simulink model "sm_car"  (R2025a)
settings: Solver=ode23t  StartTime=0.0  StopTime=400  MaxStep=0.4  RelTol=1e-3  AbsTol=1e-3  EnableMultiTasking=on
PreLoadFcn:
  | % Due to usability issue in Repeating Sequence block
  | warning('off','Simulink:Masking:Invalid');
  | 
  | % Eliminate unnecessary warnings in inactive variants
  | % Warnings generated only if you click through inactive variant
  | warning('off','MATLAB:nonExistentField');
  | warning('off','Simulink:Parameters:BlkParamUndefined');
PostLoadFcn:
  | set_param([bdroot '/Vehicle'],'popup_trailer','Off')
  | warning('off','sm:sli:setup:compile:LocalSolverNotSupported')
  | %sm_car_config_maneuver(bdroot,'WOT Braking');
  | sm_car_config_vehicle(bdroot,'false');
  | sm_car_config_logging(bdroot);
InitFcn:
  | sm_car_config_camera;
  | Vehicle = sm_car_vehcfg_checkConfig(Vehicle);
  | sm_car_check_tire_model(bdroot);
StartFcn:
  | tic;
StopFcn:
  | Elapsed_Sim_Time = toc;
  | % disp(['Elapsed Sim Time = ' num2str(Elapsed_Sim_Time)]);
undefined symbols (not defined in the file): Axle1D, AxleIn, Camera, Control, Driver, Free, Init, Maneuver, Pedal, RaceFix, RaceSpin, Scene, ShaftL1, ShaftL2, ShaftR1, ShaftR2, Soft, Stiff, Visual, X, xy_data_car_side, Y, Z
libraries: sm_lib x1546, nesl_utility x528, fl_lib x480, SimscapeFluids_lib x61, sdl_lib x49, simulink x29, ee_lib x7, simulink_extras x6, Linkage_Systems x4, Tire_1x2x x4, AntiRollBar_Systems x2, Linkage_Decoupled x2
(part 3 of 79)

== system sm_car/Camera Frames/Transform FR ==
  Transform Camera Frame : sm_lib/Frames and Transforms/Rigid Transform  RotationMethod=RotationSequence  FollAlignAxisA=+X  BaseAlignAxisA=+Y  FollAlignAxisB=+Y  BaseAlignAxisB=+Z  RotationStandardAxis=+Z  RotationAngle=0.0  RotationAngleUnits=deg  RotationArbitraryAxis=[0 0 1]  RotationSequenceAxes=FollowerAxes  RotationSequence=ZYX  RotationSequenceAngles=CF.a.Value(3:-1:1)  RotationSequenceAnglesUnits=deg  RotationMatrix=[1 0 0; 0 1 0; 0 0 1]  Quaternion=[1 0 0 0]  TranslationMethod=Cartesian  TranslationCartesianOffset=CF.s.Value  TranslationCartesianOffsetUnits=m  TranslationStandardAxis=+Z  TranslationStandardOffset=0  TranslationStandardOffsetUnits=m  TranslationROffset=0  TranslationROffsetUnits=m  TranslationThetaOffset=0  TranslationThetaOffsetUnits=deg  TranslationZOffset=0  TranslationZOffsetUnits=m
  B : PMIOPort  Side=Left
  F : PMIOPort  Port=2  Side=Right
  connections:
  Transform Camera Frame/RConn1 -- F/RConn1
  Transform Camera Frame/LConn1 -- B/RConn1

== system sm_car/Camera Frames/Transform FixO FL ==
  Transform Camera Frame : sm_lib/Frames and Transforms/Rigid Transform  RotationMethod=RotationSequence  FollAlignAxisA=+X  BaseAlignAxisA=+Y  FollAlignAxisB=+Y  BaseAlignAxisB=+Z  RotationStandardAxis=+Z  RotationAngle=0.0  RotationAngleUnits=deg  RotationArbitraryAxis=[0 0 1]  RotationSequenceAxes=FollowerAxes  RotationSequence=ZYX  RotationSequenceAngles=CF.a.Value(3:-1:1)  RotationSequenceAnglesUnits=deg  RotationMatrix=[1 0 0; 0 1 0; 0 0 1]  Quaternion=[1 0 0 0]  TranslationMethod=Cartesian  TranslationCartesianOffset=CF.s.Value  TranslationCartesianOffsetUnits=m  TranslationStandardAxis=+Z  TranslationStandardOffset=0  TranslationStandardOffsetUnits=m  TranslationROffset=0  TranslationROffsetUnits=m  TranslationThetaOffset=0  TranslationThetaOffsetUnits=deg  TranslationZOffset=0  TranslationZOffsetUnits=m
  B : PMIOPort  Side=Left
  F : PMIOPort  Port=2  Side=Right
  connections:
  Transform Camera Frame/RConn1 -- F/RConn1
  Transform Camera Frame/LConn1 -- B/RConn1

== system sm_car/Camera Frames/Transform FixO FR ==
  Transform Camera Frame : sm_lib/Frames and Transforms/Rigid Transform  RotationMethod=RotationSequence  FollAlignAxisA=+X  BaseAlignAxisA=+Y  FollAlignAxisB=+Y  BaseAlignAxisB=+Z  RotationStandardAxis=+Z  RotationAngle=0.0  RotationAngleUnits=deg  RotationArbitraryAxis=[0 0 1]  RotationSequenceAxes=FollowerAxes  RotationSequence=ZYX  RotationSequenceAngles=CF.a.Value(3:-1:1)  RotationSequenceAnglesUnits=deg  RotationMatrix=[1 0 0; 0 1 0; 0 0 1]  Quaternion=[1 0 0 0]  TranslationMethod=Cartesian  TranslationCartesianOffset=CF.s.Value  TranslationCartesianOffsetUnits=m  TranslationStandardAxis=+Z  TranslationStandardOffset=0  TranslationStandardOffsetUnits=m  TranslationROffset=0  TranslationROffsetUnits=m  TranslationThetaOffset=0  TranslationThetaOffsetUnits=deg  TranslationZOffset=0  TranslationZOffsetUnits=m
  B : PMIOPort  Side=Left
  F : PMIOPort  Port=2  Side=Right
  connections:
  Transform Camera Frame/RConn1 -- F/RConn1
  Transform Camera Frame/LConn1 -- B/RConn1

== system sm_car/Camera Frames/Transform FixO Front ==
  Transform Camera Frame : sm_lib/Frames and Transforms/Rigid Transform  RotationMethod=RotationSequence  FollAlignAxisA=+X  BaseAlignAxisA=+Y  FollAlignAxisB=+Y  BaseAlignAxisB=+Z  RotationStandardAxis=+Z  RotationAngle=0.0  RotationAngleUnits=deg  RotationArbitraryAxis=[0 0 1]  RotationSequenceAxes=FollowerAxes  RotationSequence=ZYX  RotationSequenceAngles=CF.a.Value(3:-1:1)  RotationSequenceAnglesUnits=deg  RotationMatrix=[1 0 0; 0 1 0; 0 0 1]  Quaternion=[1 0 0 0]  TranslationMethod=Cartesian  TranslationCartesianOffset=CF.s.Value  TranslationCartesianOffsetUnits=m  TranslationStandardAxis=+Z  TranslationStandardOffset=0  TranslationStandardOffsetUnits=m  TranslationROffset=0  TranslationROffsetUnits=m  TranslationThetaOffset=0  TranslationThetaOffsetUnits=deg  TranslationZOffset=0  TranslationZOffsetUnits=m
  B : PMIOPort  Side=Left
  F : PMIOPort  Port=2  Side=Right
  connections:
  Transform Camera Frame/RConn1 -- F/RConn1
  Transform Camera Frame/LConn1 -- B/RConn1

== system sm_car/Camera Frames/Transform FixO Left ==
  Transform Camera Frame : sm_lib/Frames and Transforms/Rigid Transform  RotationMethod=RotationSequence  FollAlignAxisA=+X  BaseAlignAxisA=+Y  FollAlignAxisB=+Y  BaseAlignAxisB=+Z  RotationStandardAxis=+Z  RotationAngle=0.0  RotationAngleUnits=deg  RotationArbitraryAxis=[0 0 1]  RotationSequenceAxes=FollowerAxes  RotationSequence=ZYX  RotationSequenceAngles=CF.a.Value(3:-1:1)  RotationSequenceAnglesUnits=deg  RotationMatrix=[1 0 0; 0 1 0; 0 0 1]  Quaternion=[1 0 0 0]  TranslationMethod=Cartesian  TranslationCartesianOffset=CF.s.Value  TranslationCartesianOffsetUnits=m  TranslationStandardAxis=+Z  TranslationStandardOffset=0  TranslationStandardOffsetUnits=m  TranslationROffset=0  TranslationROffsetUnits=m  TranslationThetaOffset=0  TranslationThetaOffsetUnits=deg  TranslationZOffset=0  TranslationZOffsetUnits=m
  B : PMIOPort  Side=Left
  F : PMIOPort  Port=2  Side=Right
  connections:
  Transform Camera Frame/RConn1 -- F/RConn1
  Transform Camera Frame/LConn1 -- B/RConn1

== system sm_car/Camera Frames/Transform FixO RL ==
  Transform Camera Frame : sm_lib/Frames and Transforms/Rigid Transform  RotationMethod=RotationSequence  FollAlignAxisA=+X  BaseAlignAxisA=+Y  FollAlignAxisB=+Y  BaseAlignAxisB=+Z  RotationStandardAxis=+Z  RotationAngle=0.0  RotationAngleUnits=deg  RotationArbitraryAxis=[0 0 1]  RotationSequenceAxes=FollowerAxes  RotationSequence=ZYX  RotationSequenceAngles=CF.a.Value(3:-1:1)  RotationSequenceAnglesUnits=deg  RotationMatrix=[1 0 0; 0 1 0; 0 0 1]  Quaternion=[1 0 0 0]  TranslationMethod=Cartesian  TranslationCartesianOffset=CF.s.Value  TranslationCartesianOffsetUnits=m  TranslationStandardAxis=+Z  TranslationStandardOffset=0  TranslationStandardOffsetUnits=m  TranslationROffset=0  TranslationROffsetUnits=m  TranslationThetaOffset=0  TranslationThetaOffsetUnits=deg  TranslationZOffset=0  TranslationZOffsetUnits=m
  B : PMIOPort  Side=Left
  F : PMIOPort  Port=2  Side=Right
  connections:
  Transform Camera Frame/RConn1 -- F/RConn1
  Transform Camera Frame/LConn1 -- B/RConn1

== system sm_car/Camera Frames/Transform FixO RR ==
  Transform Camera Frame : sm_lib/Frames and Transforms/Rigid Transform  RotationMethod=RotationSequence  FollAlignAxisA=+X  BaseAlignAxisA=+Y  FollAlignAxisB=+Y  BaseAlignAxisB=+Z  RotationStandardAxis=+Z  RotationAngle=0.0  RotationAngleUnits=deg  RotationArbitraryAxis=[0 0 1]  RotationSequenceAxes=FollowerAxes  RotationSequence=ZYX  RotationSequenceAngles=CF.a.Value(3:-1:1)  RotationSequenceAnglesUnits=deg  RotationMatrix=[1 0 0; 0 1 0; 0 0 1]  Quaternion=[1 0 0 0]  TranslationMethod=Cartesian  TranslationCartesianOffset=CF.s.Value  TranslationCartesianOffsetUnits=m  TranslationStandardAxis=+Z  TranslationStandardOffset=0  TranslationStandardOffsetUnits=m  TranslationROffset=0  TranslationROffsetUnits=m  TranslationThetaOffset=0  TranslationThetaOffsetUnits=deg  TranslationZOffset=0  TranslationZOffsetUnits=m
  B : PMIOPort  Side=Left
  F : PMIOPort  Port=2  Side=Right
  connections:
  Transform Camera Frame/RConn1 -- F/RConn1
  Transform Camera Frame/LConn1 -- B/RConn1

== system sm_car/Camera Frames/Transform FixO Rear ==
  Transform Camera Frame : sm_lib/Frames and Transforms/Rigid Transform  RotationMethod=RotationSequence  FollAlignAxisA=+X  BaseAlignAxisA=+Y  FollAlignAxisB=+Y  BaseAlignAxisB=+Z  RotationStandardAxis=+Z  RotationAngle=0.0  RotationAngleUnits=deg  RotationArbitraryAxis=[0 0 1]  RotationSequenceAxes=FollowerAxes  RotationSequence=ZYX  RotationSequenceAngles=CF.a.Value(3:-1:1)  RotationSequenceAnglesUnits=deg  RotationMatrix=[1 0 0; 0 1 0; 0 0 1]  Quaternion=[1 0 0 0]  TranslationMethod=Cartesian  TranslationCartesianOffset=CF.s.Value  TranslationCartesianOffsetUnits=m  TranslationStandardAxis=+Z  TranslationStandardOffset=0  TranslationStandardOffsetUnits=m  TranslationROffset=0  TranslationROffsetUnits=m  TranslationThetaOffset=0  TranslationThetaOffsetUnits=deg  TranslationZOffset=0  TranslationZOffsetUnits=m
  B : PMIOPort  Side=Left
  F : PMIOPort  Port=2  Side=Right
  connections:
  Transform Camera Frame/RConn1 -- F/RConn1
  Transform Camera Frame/LConn1 -- B/RConn1

== system sm_car/Camera Frames/Transform FixO Right ==
  Transform Camera Frame : sm_lib/Frames and Transforms/Rigid Transform  RotationMethod=RotationSequence  FollAlignAxisA=+X  BaseAlignAxisA=+Y  FollAlignAxisB=+Y  BaseAlignAxisB=+Z  RotationStandardAxis=+Z  RotationAngle=0.0  RotationAngleUnits=deg  RotationArbitraryAxis=[0 0 1]  RotationSequenceAxes=FollowerAxes  RotationSequence=ZYX  RotationSequenceAngles=CF.a.Value(3:-1:1)  RotationSequenceAnglesUnits=deg  RotationMatrix=[1 0 0; 0 1 0; 0 0 1]  Quaternion=[1 0 0 0]  TranslationMethod=Cartesian  TranslationCartesianOffset=CF.s.Value  TranslationCartesianOffsetUnits=m  TranslationStandardAxis=+Z  TranslationStandardOffset=0  TranslationStandardOffsetUnits=m  TranslationROffset=0  TranslationROffsetUnits=m  TranslationThetaOffset=0  TranslationThetaOffsetUnits=deg  TranslationZOffset=0  TranslationZOffsetUnits=m
  B : PMIOPort  Side=Left
  F : PMIOPort  Port=2  Side=Right
  connections:
  Transform Camera Frame/RConn1 -- F/RConn1
  Transform Camera Frame/LConn1 -- B/RConn1

== system sm_car/Camera Frames/Transform FixO Top ==
  Transform Camera Frame : sm_lib/Frames and Transforms/Rigid Transform  RotationMethod=RotationSequence  FollAlignAxisA=+X  BaseAlignAxisA=+Y  FollAlignAxisB=+Y  BaseAlignAxisB=+Z  RotationStandardAxis=+Z  RotationAngle=0.0  RotationAngleUnits=deg  RotationArbitraryAxis=[0 0 1]  RotationSequenceAxes=FollowerAxes  RotationSequence=ZYX  RotationSequenceAngles=CF.a.Value(3:-1:1)  RotationSequenceAnglesUnits=deg  RotationMatrix=[1 0 0; 0 1 0; 0 0 1]  Quaternion=[1 0 0 0]  TranslationMethod=Cartesian  TranslationCartesianOffset=CF.s.Value  TranslationCartesianOffsetUnits=m  TranslationStandardAxis=+Z  TranslationStandardOffset=0  TranslationStandardOffsetUnits=m  TranslationROffset=0  TranslationROffsetUnits=m  TranslationThetaOffset=0  TranslationThetaOffsetUnits=deg  TranslationZOffset=0  TranslationZOffsetUnits=m
  B : PMIOPort  Side=Left
  F : PMIOPort  Port=2  Side=Right
  connections:
  Transform Camera Frame/RConn1 -- F/RConn1
  Transform Camera Frame/LConn1 -- B/RConn1

== system sm_car/Camera Frames/Transform Front ==
  Transform Camera Frame : sm_lib/Frames and Transforms/Rigid Transform  RotationMethod=RotationSequence  FollAlignAxisA=+X  BaseAlignAxisA=+Y  FollAlignAxisB=+Y  BaseAlignAxisB=+Z  RotationStandardAxis=+Z  RotationAngle=0.0  RotationAngleUnits=deg  RotationArbitraryAxis=[0 0 1]  RotationSequenceAxes=FollowerAxes  RotationSequence=ZYX  RotationSequenceAngles=CF.a.Value(3:-1:1)  RotationSequenceAnglesUnits=deg  RotationMatrix=[1 0 0; 0 1 0; 0 0 1]  Quaternion=[1 0 0 0]  TranslationMethod=Cartesian  TranslationCartesianOffset=CF.s.Value  TranslationCartesianOffsetUnits=m  TranslationStandardAxis=+Z  TranslationStandardOffset=0  TranslationStandardOffsetUnits=m  TranslationROffset=0  TranslationROffsetUnits=m  TranslationThetaOffset=0  TranslationThetaOffsetUnits=deg  TranslationZOffset=0  TranslationZOffsetUnits=m
  B : PMIOPort  Side=Left
  F : PMIOPort  Port=2  Side=Right
  connections:
  Transform Camera Frame/RConn1 -- F/RConn1
  Transform Camera Frame/LConn1 -- B/RConn1

== system sm_car/Camera Frames/Transform Left ==
  Transform Camera Frame : sm_lib/Frames and Transforms/Rigid Transform  RotationMethod=RotationSequence  FollAlignAxisA=+X  BaseAlignAxisA=+Y  FollAlignAxisB=+Y  BaseAlignAxisB=+Z  RotationStandardAxis=+Z  RotationAngle=0.0  RotationAngleUnits=deg  RotationArbitraryAxis=[0 0 1]  RotationSequenceAxes=FollowerAxes  RotationSequence=ZYX  RotationSequenceAngles=CF.a.Value(3:-1:1)  RotationSequenceAnglesUnits=deg  RotationMatrix=[1 0 0; 0 1 0; 0 0 1]  Quaternion=[1 0 0 0]  TranslationMethod=Cartesian  TranslationCartesianOffset=CF.s.Value  TranslationCartesianOffsetUnits=m  TranslationStandardAxis=+Z  TranslationStandardOffset=0  TranslationStandardOffsetUnits=m  TranslationROffset=0  TranslationROffsetUnits=m  TranslationThetaOffset=0  TranslationThetaOffsetUnits=deg  TranslationZOffset=0  TranslationZOffsetUnits=m
  B : PMIOPort  Side=Left
  F : PMIOPort  Port=2  Side=Right
  connections:
  Transform Camera Frame/RConn1 -- F/RConn1
  Transform Camera Frame/LConn1 -- B/RConn1

== system sm_car/Camera Frames/Transform RL ==
  Transform Camera Frame : sm_lib/Frames and Transforms/Rigid Transform  RotationMethod=RotationSequence  FollAlignAxisA=+X  BaseAlignAxisA=+Y  FollAlignAxisB=+Y  BaseAlignAxisB=+Z  RotationStandardAxis=+Z  RotationAngle=0.0  RotationAngleUnits=deg  RotationArbitraryAxis=[0 0 1]  RotationSequenceAxes=FollowerAxes  RotationSequence=ZYX  RotationSequenceAngles=CF.a.Value(3:-1:1)  RotationSequenceAnglesUnits=deg  RotationMatrix=[1 0 0; 0 1 0; 0 0 1]  Quaternion=[1 0 0 0]  TranslationMethod=Cartesian  TranslationCartesianOffset=CF.s.Value  TranslationCartesianOffsetUnits=m  TranslationStandardAxis=+Z  TranslationStandardOffset=0  TranslationStandardOffsetUnits=m  TranslationROffset=0  TranslationROffsetUnits=m  TranslationThetaOffset=0  TranslationThetaOffsetUnits=deg  TranslationZOffset=0  TranslationZOffsetUnits=m
  B : PMIOPort  Side=Left
  F : PMIOPort  Port=2  Side=Right
  connections:
  Transform Camera Frame/RConn1 -- F/RConn1
  Transform Camera Frame/LConn1 -- B/RConn1

== system sm_car/Camera Frames/Transform RR ==
  Transform Camera Frame : sm_lib/Frames and Transforms/Rigid Transform  RotationMethod=RotationSequence  FollAlignAxisA=+X  BaseAlignAxisA=+Y  FollAlignAxisB=+Y  BaseAlignAxisB=+Z  RotationStandardAxis=+Z  RotationAngle=0.0  RotationAngleUnits=deg  RotationArbitraryAxis=[0 0 1]  RotationSequenceAxes=FollowerAxes  RotationSequence=ZYX  RotationSequenceAngles=CF.a.Value(3:-1:1)  RotationSequenceAnglesUnits=deg  RotationMatrix=[1 0 0; 0 1 0; 0 0 1]  Quaternion=[1 0 0 0]  TranslationMethod=Cartesian  TranslationCartesianOffset=CF.s.Value  TranslationCartesianOffsetUnits=m  TranslationStandardAxis=+Z  TranslationStandardOffset=0  TranslationStandardOffsetUnits=m  TranslationROffset=0  TranslationROffsetUnits=m  TranslationThetaOffset=0  TranslationThetaOffsetUnits=deg  TranslationZOffset=0  TranslationZOffsetUnits=m
  B : PMIOPort  Side=Left
  F : PMIOPort  Port=2  Side=Right
  connections:
  Transform Camera Frame/RConn1 -- F/RConn1
  Transform Camera Frame/LConn1 -- B/RConn1

== system sm_car/Camera Frames/Transform Rear ==
  Transform Camera Frame : sm_lib/Frames and Transforms/Rigid Transform  RotationMethod=RotationSequence  FollAlignAxisA=+X  BaseAlignAxisA=+Y  FollAlignAxisB=+Y  BaseAlignAxisB=+Z  RotationStandardAxis=+Z  RotationAngle=0.0  RotationAngleUnits=deg  RotationArbitraryAxis=[0 0 1]  RotationSequenceAxes=FollowerAxes  RotationSequence=ZYX  RotationSequenceAngles=CF.a.Value(3:-1:1)  RotationSequenceAnglesUnits=deg  RotationMatrix=[1 0 0; 0 1 0; 0 0 1]  Quaternion=[1 0 0 0]  TranslationMethod=Cartesian  TranslationCartesianOffset=CF.s.Value  TranslationCartesianOffsetUnits=m  TranslationStandardAxis=+Z  TranslationStandardOffset=0  TranslationStandardOffsetUnits=m  TranslationROffset=0  TranslationROffsetUnits=m  TranslationThetaOffset=0  TranslationThetaOffsetUnits=deg  TranslationZOffset=0  TranslationZOffsetUnits=m
  B : PMIOPort  Side=Left
  F : PMIOPort  Port=2  Side=Right
  connections:
  Transform Camera Frame/RConn1 -- F/RConn1
  Transform Camera Frame/LConn1 -- B/RConn1

== system sm_car/Camera Frames/Transform Right ==
  Transform Camera Frame : sm_lib/Frames and Transforms/Rigid Transform  RotationMethod=RotationSequence  FollAlignAxisA=+X  BaseAlignAxisA=+Y  FollAlignAxisB=+Y  BaseAlignAxisB=+Z  RotationStandardAxis=+Z  RotationAngle=0.0  RotationAngleUnits=deg  RotationArbitraryAxis=[0 0 1]  RotationSequenceAxes=FollowerAxes  RotationSequence=ZYX  RotationSequenceAngles=CF.a.Value(3:-1:1)  RotationSequenceAnglesUnits=deg  RotationMatrix=[1 0 0; 0 1 0; 0 0 1]  Quaternion=[1 0 0 0]  TranslationMethod=Cartesian  TranslationCartesianOffset=CF.s.Value  TranslationCartesianOffsetUnits=m  TranslationStandardAxis=+Z  TranslationStandardOffset=0  TranslationStandardOffsetUnits=m  TranslationROffset=0  TranslationROffsetUnits=m  TranslationThetaOffset=0  TranslationThetaOffsetUnits=deg  TranslationZOffset=0  TranslationZOffsetUnits=m
  B : PMIOPort  Side=Left
  F : PMIOPort  Port=2  Side=Right
  connections:
  Transform Camera Frame/RConn1 -- F/RConn1
  Transform Camera Frame/LConn1 -- B/RConn1

== system sm_car/Camera Frames/Transform SuspF ==
  Transform Camera Frame : sm_lib/Frames and Transforms/Rigid Transform  RotationMethod=RotationSequence  FollAlignAxisA=+X  BaseAlignAxisA=+Y  FollAlignAxisB=+Y  BaseAlignAxisB=+Z  RotationStandardAxis=+Z  RotationAngle=0.0  RotationAngleUnits=deg  RotationArbitraryAxis=[0 0 1]  RotationSequenceAxes=FollowerAxes  RotationSequence=ZYX  RotationSequenceAngles=CF.a.Value(3:-1:1)  RotationSequenceAnglesUnits=deg  RotationMatrix=[1 0 0; 0 1 0; 0 0 1]  Quaternion=[1 0 0 0]  TranslationMethod=Cartesian  TranslationCartesianOffset=CF.s.Value  TranslationCartesianOffsetUnits=m  TranslationStandardAxis=+Z  TranslationStandardOffset=0  TranslationStandardOffsetUnits=m  TranslationROffset=0  TranslationROffsetUnits=m  TranslationThetaOffset=0  TranslationThetaOffsetUnits=deg  TranslationZOffset=0  TranslationZOffsetUnits=m
  B : PMIOPort  Side=Left
  F : PMIOPort  Port=2  Side=Right
  connections:
  Transform Camera Frame/RConn1 -- F/RConn1
  Transform Camera Frame/LConn1 -- B/RConn1

== system sm_car/Camera Frames/Transform SuspR ==
  Transform Camera Frame : sm_lib/Frames and Transforms/Rigid Transform  RotationMethod=RotationSequence  FollAlignAxisA=+X  BaseAlignAxisA=+Y  FollAlignAxisB=+Y  BaseAlignAxisB=+Z  RotationStandardAxis=+Z  RotationAngle=0.0  RotationAngleUnits=deg  RotationArbitraryAxis=[0 0 1]  RotationSequenceAxes=FollowerAxes  RotationSequence=ZYX  RotationSequenceAngles=CF.a.Value(3:-1:1)  RotationSequenceAnglesUnits=deg  RotationMatrix=[1 0 0; 0 1 0; 0 0 1]  Quaternion=[1 0 0 0]  TranslationMethod=Cartesian  TranslationCartesianOffset=CF.s.Value  TranslationCartesianOffsetUnits=m  TranslationStandardAxis=+Z  TranslationStandardOffset=0  TranslationStandardOffsetUnits=m  TranslationROffset=0  TranslationROffsetUnits=m  TranslationThetaOffset=0  TranslationThetaOffsetUnits=deg  TranslationZOffset=0  TranslationZOffsetUnits=m
  B : PMIOPort  Side=Left
  F : PMIOPort  Port=2  Side=Right
  connections:
  Transform Camera Frame/RConn1 -- F/RConn1
  Transform Camera Frame/LConn1 -- B/RConn1

== system sm_car/Camera Frames/Transform Top ==
  Transform Camera Frame : sm_lib/Frames and Transforms/Rigid Transform  RotationMethod=RotationSequence  FollAlignAxisA=+X  BaseAlignAxisA=+Y  FollAlignAxisB=+Y  BaseAlignAxisB=+Z  RotationStandardAxis=+Z  RotationAngle=0.0  RotationAngleUnits=deg  RotationArbitraryAxis=[0 0 1]  RotationSequenceAxes=FollowerAxes  RotationSequence=ZYX  RotationSequenceAngles=CF.a.Value(3:-1:1)  RotationSequenceAnglesUnits=deg  RotationMatrix=[1 0 0; 0 1 0; 0 0 1]  Quaternion=[1 0 0 0]  TranslationMethod=Cartesian  TranslationCartesianOffset=CF.s.Value  TranslationCartesianOffsetUnits=m  TranslationStandardAxis=+Z  TranslationStandardOffset=0  TranslationStandardOffsetUnits=m  TranslationROffset=0  TranslationROffsetUnits=m  TranslationThetaOffset=0  TranslationThetaOffsetUnits=deg  TranslationZOffset=0  TranslationZOffsetUnits=m
  B : PMIOPort  Side=Left
  F : PMIOPort  Port=2  Side=Right
  connections:
  Transform Camera Frame/RConn1 -- F/RConn1
  Transform Camera Frame/LConn1 -- B/RConn1

== system sm_car/Camera Frames/Transform View Seat FL ==
  Transform Camera Frame : sm_lib/Frames and Transforms/Rigid Transform  RotationMethod=RotationSequence  FollAlignAxisA=+X  BaseAlignAxisA=+Y  FollAlignAxisB=+Y  BaseAlignAxisB=+Z  RotationStandardAxis=+Z  RotationAngle=0.0  RotationAngleUnits=deg  RotationArbitraryAxis=[0 0 1]  RotationSequenceAxes=FollowerAxes  RotationSequence=ZYX  RotationSequenceAngles=CF.a.Value(3:-1:1)  RotationSequenceAnglesUnits=deg  RotationMatrix=[1 0 0; 0 1 0; 0 0 1]  Quaternion=[1 0 0 0]  TranslationMethod=Cartesian  TranslationCartesianOffset=CF.s.Value  TranslationCartesianOffsetUnits=m  TranslationStandardAxis=+Z  TranslationStandardOffset=0  TranslationStandardOffsetUnits=m  TranslationROffset=0  TranslationROffsetUnits=m  TranslationThetaOffset=0  TranslationThetaOffsetUnits=deg  TranslationZOffset=0  TranslationZOffsetUnits=m
  B : PMIOPort  Side=Left
  F : PMIOPort  Port=2  Side=Right
  connections:
  Transform Camera Frame/RConn1 -- F/RConn1
  Transform Camera Frame/LConn1 -- B/RConn1

== system sm_car/Camera Frames/Transform View Seat FR ==
  Transform Camera Frame : sm_lib/Frames and Transforms/Rigid Transform  RotationMethod=RotationSequence  FollAlignAxisA=+X  BaseAlignAxisA=+Y  FollAlignAxisB=+Y  BaseAlignAxisB=+Z  RotationStandardAxis=+Z  RotationAngle=0.0  RotationAngleUnits=deg  RotationArbitraryAxis=[0 0 1]  RotationSequenceAxes=FollowerAxes  RotationSequence=ZYX  RotationSequenceAngles=CF.a.Value(3:-1:1)  RotationSequenceAnglesUnits=deg  RotationMatrix=[1 0 0; 0 1 0; 0 0 1]  Quaternion=[1 0 0 0]  TranslationMethod=Cartesian  TranslationCartesianOffset=CF.s.Value  TranslationCartesianOffsetUnits=m  TranslationStandardAxis=+Z  TranslationStandardOffset=0  TranslationStandardOffsetUnits=m  TranslationROffset=0  TranslationROffsetUnits=m  TranslationThetaOffset=0  TranslationThetaOffsetUnits=deg  TranslationZOffset=0  TranslationZOffsetUnits=m
  B : PMIOPort  Side=Left
  F : PMIOPort  Port=2  Side=Right
  connections:
  Transform Camera Frame/RConn1 -- F/RConn1
  Transform Camera Frame/LConn1 -- B/RConn1

== system sm_car/Camera Frames/Transform View Susp FL ==
  Transform Camera Frame : sm_lib/Frames and Transforms/Rigid Transform  RotationMethod=RotationSequence  FollAlignAxisA=+X  BaseAlignAxisA=+Y  FollAlignAxisB=+Y  BaseAlignAxisB=+Z  RotationStandardAxis=+Z  RotationAngle=0.0  RotationAngleUnits=deg  RotationArbitraryAxis=[0 0 1]  RotationSequenceAxes=FollowerAxes  RotationSequence=ZYX  RotationSequenceAngles=CF.a.Value(3:-1:1)  RotationSequenceAnglesUnits=deg  RotationMatrix=[1 0 0; 0 1 0; 0 0 1]  Quaternion=[1 0 0 0]  TranslationMethod=Cartesian  TranslationCartesianOffset=CF.s.Value  TranslationCartesianOffsetUnits=m  TranslationStandardAxis=+Z  TranslationStandardOffset=0  TranslationStandardOffsetUnits=m  TranslationROffset=0  TranslationROffsetUnits=m  TranslationThetaOffset=0  TranslationThetaOffsetUnits=deg  TranslationZOffset=0  TranslationZOffsetUnits=m
  B : PMIOPort  Side=Left
  F : PMIOPort  Port=2  Side=Right
  connections:
  Transform Camera Frame/RConn1 -- F/RConn1
  Transform Camera Frame/LConn1 -- B/RConn1

== system sm_car/Camera Frames/Transform View Susp FR ==
  Transform Camera Frame : sm_lib/Frames and Transforms/Rigid Transform  RotationMethod=RotationSequence  FollAlignAxisA=+X  BaseAlignAxisA=+Y  FollAlignAxisB=+Y  BaseAlignAxisB=+Z  RotationStandardAxis=+Z  RotationAngle=0.0  RotationAngleUnits=deg  RotationArbitraryAxis=[0 0 1]  RotationSequenceAxes=FollowerAxes  RotationSequence=ZYX  RotationSequenceAngles=CF.a.Value(3:-1:1)  RotationSequenceAnglesUnits=deg  RotationMatrix=[1 0 0; 0 1 0; 0 0 1]  Quaternion=[1 0 0 0]  TranslationMethod=Cartesian  TranslationCartesianOffset=CF.s.Value  TranslationCartesianOffsetUnits=m  TranslationStandardAxis=+Z  TranslationStandardOffset=0  TranslationStandardOffsetUnits=m  TranslationROffset=0  TranslationROffsetUnits=m  TranslationThetaOffset=0  TranslationThetaOffsetUnits=deg  TranslationZOffset=0  TranslationZOffsetUnits=m
  B : PMIOPort  Side=Left
  F : PMIOPort  Port=2  Side=Right
  connections:
  Transform Camera Frame/RConn1 -- F/RConn1
  Transform Camera Frame/LConn1 -- B/RConn1

== system sm_car/Camera Frames/Transform View Susp RL ==
  Transform Camera Frame : sm_lib/Frames and Transforms/Rigid Transform  RotationMethod=RotationSequence  FollAlignAxisA=+X  BaseAlignAxisA=+Y  FollAlignAxisB=+Y  BaseAlignAxisB=+Z  RotationStandardAxis=+Z  RotationAngle=0.0  RotationAngleUnits=deg  RotationArbitraryAxis=[0 0 1]  RotationSequenceAxes=FollowerAxes  RotationSequence=ZYX  RotationSequenceAngles=CF.a.Value(3:-1:1)  RotationSequenceAnglesUnits=deg  RotationMatrix=[1 0 0; 0 1 0; 0 0 1]  Quaternion=[1 0 0 0]  TranslationMethod=Cartesian  TranslationCartesianOffset=CF.s.Value  TranslationCartesianOffsetUnits=m  TranslationStandardAxis=+Z  TranslationStandardOffset=0  TranslationStandardOffsetUnits=m  TranslationROffset=0  TranslationROffsetUnits=m  TranslationThetaOffset=0  TranslationThetaOffsetUnits=deg  TranslationZOffset=0  TranslationZOffsetUnits=m
  B : PMIOPort  Side=Left
  F : PMIOPort  Port=2  Side=Right
  connections:
  Transform Camera Frame/RConn1 -- F/RConn1
  Transform Camera Frame/LConn1 -- B/RConn1

== system sm_car/Camera Frames/Transform View Susp RR ==
  Transform Camera Frame : sm_lib/Frames and Transforms/Rigid Transform  RotationMethod=RotationSequence  FollAlignAxisA=+X  BaseAlignAxisA=+Y  FollAlignAxisB=+Y  BaseAlignAxisB=+Z  RotationStandardAxis=+Z  RotationAngle=0.0  RotationAngleUnits=deg  RotationArbitraryAxis=[0 0 1]  RotationSequenceAxes=FollowerAxes  RotationSequence=ZYX  RotationSequenceAngles=CF.a.Value(3:-1:1)  RotationSequenceAnglesUnits=deg  RotationMatrix=[1 0 0; 0 1 0; 0 0 1]  Quaternion=[1 0 0 0]  TranslationMethod=Cartesian  TranslationCartesianOffset=CF.s.Value  TranslationCartesianOffsetUnits=m  TranslationStandardAxis=+Z  TranslationStandardOffset=0  TranslationStandardOffsetUnits=m  TranslationROffset=0  TranslationROffsetUnits=m  TranslationThetaOffset=0  TranslationThetaOffsetUnits=deg  TranslationZOffset=0  TranslationZOffsetUnits=m
  B : PMIOPort  Side=Left
  F : PMIOPort  Port=2  Side=Right
  connections:
  Transform Camera Frame/RConn1 -- F/RConn1
  Transform Camera Frame/LConn1 -- B/RConn1

== system sm_car/Camera Frames/Transform Wheel FL ==
  Transform Camera Frame : sm_lib/Frames and Transforms/Rigid Transform  RotationMethod=RotationSequence  FollAlignAxisA=+X  BaseAlignAxisA=+Y  FollAlignAxisB=+Y  BaseAlignAxisB=+Z  RotationStandardAxis=+Z  RotationAngle=0.0  RotationAngleUnits=deg  RotationArbitraryAxis=[0 0 1]  RotationSequenceAxes=FollowerAxes  RotationSequence=ZYX  RotationSequenceAngles=CF.a.Value(3:-1:1)  RotationSequenceAnglesUnits=deg  RotationMatrix=[1 0 0; 0 1 0; 0 0 1]  Quaternion=[1 0 0 0]  TranslationMethod=Cartesian  TranslationCartesianOffset=CF.s.Value  TranslationCartesianOffsetUnits=m  TranslationStandardAxis=+Z  TranslationStandardOffset=0  TranslationStandardOffsetUnits=m  TranslationROffset=0  TranslationROffsetUnits=m  TranslationThetaOffset=0  TranslationThetaOffsetUnits=deg  TranslationZOffset=0  TranslationZOffsetUnits=m
  B : PMIOPort  Side=Left
  F : PMIOPort  Port=2  Side=Right
  connections:
  Transform Camera Frame/RConn1 -- F/RConn1
  Transform Camera Frame/LConn1 -- B/RConn1

== system sm_car/Camera Frames/Transform Wheel FR ==
  Transform Camera Frame : sm_lib/Frames and Transforms/Rigid Transform  RotationMethod=RotationSequence  FollAlignAxisA=+X  BaseAlignAxisA=+Y  FollAlignAxisB=+Y  BaseAlignAxisB=+Z  RotationStandardAxis=+Z  RotationAngle=0.0  RotationAngleUnits=deg  RotationArbitraryAxis=[0 0 1]  RotationSequenceAxes=FollowerAxes  RotationSequence=ZYX  RotationSequenceAngles=CF.a.Value(3:-1:1)  RotationSequenceAnglesUnits=deg  RotationMatrix=[1 0 0; 0 1 0; 0 0 1]  Quaternion=[1 0 0 0]  TranslationMethod=Cartesian  TranslationCartesianOffset=CF.s.Value  TranslationCartesianOffsetUnits=m  TranslationStandardAxis=+Z  TranslationStandardOffset=0  TranslationStandardOffsetUnits=m  TranslationROffset=0  TranslationROffsetUnits=m  TranslationThetaOffset=0  TranslationThetaOffsetUnits=deg  TranslationZOffset=0  TranslationZOffsetUnits=m
  B : PMIOPort  Side=Left
  F : PMIOPort  Port=2  Side=Right
  connections:
  Transform Camera Frame/RConn1 -- F/RConn1
  Transform Camera Frame/LConn1 -- B/RConn1

== system sm_car/Camera Frames/Transform Wheel RL ==
  Transform Camera Frame : sm_lib/Frames and Transforms/Rigid Transform  RotationMethod=RotationSequence  FollAlignAxisA=+X  BaseAlignAxisA=+Y  FollAlignAxisB=+Y  BaseAlignAxisB=+Z  RotationStandardAxis=+Z  RotationAngle=0.0  RotationAngleUnits=deg  RotationArbitraryAxis=[0 0 1]  RotationSequenceAxes=FollowerAxes  RotationSequence=ZYX  RotationSequenceAngles=CF.a.Value(3:-1:1)  RotationSequenceAnglesUnits=deg  RotationMatrix=[1 0 0; 0 1 0; 0 0 1]  Quaternion=[1 0 0 0]  TranslationMethod=Cartesian  TranslationCartesianOffset=CF.s.Value  TranslationCartesianOffsetUnits=m  TranslationStandardAxis=+Z  TranslationStandardOffset=0  TranslationStandardOffsetUnits=m  TranslationROffset=0  TranslationROffsetUnits=m  TranslationThetaOffset=0  TranslationThetaOffsetUnits=deg  TranslationZOffset=0  TranslationZOffsetUnits=m
  B : PMIOPort  Side=Left
  F : PMIOPort  Port=2  Side=Right
  connections:
  Transform Camera Frame/RConn1 -- F/RConn1
  Transform Camera Frame/LConn1 -- B/RConn1

== system sm_car/Camera Frames/Transform Wheel RR ==
  Transform Camera Frame : sm_lib/Frames and Transforms/Rigid Transform  RotationMethod=RotationSequence  FollAlignAxisA=+X  BaseAlignAxisA=+Y  FollAlignAxisB=+Y  BaseAlignAxisB=+Z  RotationStandardAxis=+Z  RotationAngle=0.0  RotationAngleUnits=deg  RotationArbitraryAxis=[0 0 1]  RotationSequenceAxes=FollowerAxes  RotationSequence=ZYX  RotationSequenceAngles=CF.a.Value(3:-1:1)  RotationSequenceAnglesUnits=deg  RotationMatrix=[1 0 0; 0 1 0; 0 0 1]  Quaternion=[1 0 0 0]  TranslationMethod=Cartesian  TranslationCartesianOffset=CF.s.Value  TranslationCartesianOffsetUnits=m  TranslationStandardAxis=+Z  TranslationStandardOffset=0  TranslationStandardOffsetUnits=m  TranslationROffset=0  TranslationROffsetUnits=m  TranslationThetaOffset=0  TranslationThetaOffsetUnits=deg  TranslationZOffset=0  TranslationZOffsetUnits=m
  B : PMIOPort  Side=Left
  F : PMIOPort  Port=2  Side=Right
  connections:
  Transform Camera Frame/RConn1 -- F/RConn1
  Transform Camera Frame/LConn1 -- B/RConn1

== system sm_car/Controller/Default ==
  DrvBus : Inport
  VehBus : Inport  Port=2
  Brake Control : Subsystem  Variant=on  VariantControlMode=label  VariantControl=Variant1  LabelModeActiveChoice=Pedal  mask{popup_brake_control=Pedal, abs_tire_radiusF=Vehicle.Chassis.TireA1.tire_radius.Value, abs_tire_radiusR=Vehicle.Chassis.TireA2.tire_radius.Value}
      mask prompts: popup_brake_control "Control Type"; abs_tire_radiusF "Tire Radius Front (m)"; abs_tire_radiusR "Tire Radius Rear (m)"
      mask init:
      | set_param(gcb,'LabelModeActiveChoice',get_param(gcb,'popup_brake_control'));
      settings: AttributesFormatString=%<ActiveVariant>
      mask TypeOptions popup_brake_control: Pedal | Pressure | ABS
      mask Display: disp(' ');
  Bus Creator1 : BusCreator  Inputs=4
  Bus Creator2 : BusCreator  Inputs=4
  Bus Selector : BusSelector  OutputSignals=Chassis.Body.CG.vx
  Bus Selector1 : BusSelector  OutputSignals=aSteerWheel,rAccelPedal,rBrakePedal,Reference.vTarget
  Ctrl : Subsystem
  Damper Control : Subsystem  VariantControl=Choice  mask(Damper Control, Two Axle){popup_damper_control_A1=None, popup_damper_control_A2=None}
      mask prompts: popup_damper_control_A1 "Damper Control Axle 1"; popup_damper_control_A2 "Damper Control Axle 2"
      mask help: Configurable damper control for two axles, left and right sides.
      mask TypeOptions popup_damper_control_A1: Damper Control A1/popup_damper_control
      mask TypeOptions popup_damper_control_A2: Damper Control A2/popup_damper_control
  Driveline Control : Subsystem
  Power Control : Subsystem  mask{trq_max=Control.Default.maxTrqRequest, trq_ratio_front=Control.Default.pcnt_torque_on_f, trq_rate_up=300, trq_rate_down=-5000}
      mask prompts: trq_max "Max Torque Request"; trq_ratio_front "Ratio of Torque on Front Wheels (0-1)"; trq_rate_up "Torque Rate Limit Up (N*m/s)"; trq_rate_down "Torque Rate Limit Down (N*m/s)"
  Spring Control : Subsystem  VariantControl=Choice  mask(Spring Control, Two Axles){popup_spring_control_A1=None, popup_gas_spring_A1=Soft, popup_spring_control_A2=None, popup_gas_spring_A2=Soft}
      mask prompts: popup_spring_control_A1 "Spring Control Axle 1"; popup_gas_spring_A1 "Gas Spring (Axle 1)"; popup_spring_control_A2 "Spring Control Axle 2"; popup_gas_spring_A2 "Gas Spring (Axle 2)"
      mask help: Configurable spring control for two axles, left and right sides.
      mask TypeOptions popup_spring_control_A1: Spring Control A1/popup_spring_control
      mask Callback popup_spring_control_A1:
      | bh = gcb;
      | maskObj = Simulink.Mask.get(bh); % Get the mask object of the current block
      | psg_h   = maskObj.getParameter('popup_gas_spring_A1'); % Get the parameter to hide
      | 
      | % Check the value of ControlParam
      | controlParamValue = get_param(bh, 'popup_spring_control_A1');
      | 
      | psg_h.Visible  = 'off';
      | 
      | if strcmp(controlParamValue, 'Hydropneumatic')
      |     psg_h.Visible  = 'on';
      | else
      |     psg_h.Visible  = 'off';
      | end
      mask TypeOptions popup_gas_spring_A1: Spring Control A1/popup_gas_spring
      mask TypeOptions popup_spring_control_A2: Spring Control A2/popup_spring_control
      mask Callback popup_spring_control_A2:
      | bh = gcb;
      | maskObj = Simulink.Mask.get(bh); % Get the mask object of the current block
      | psg_h   = maskObj.getParameter('popup_gas_spring_A2'); % Get the parameter to hide
      | 
      | % Check the value of ControlParam
      | controlParamValue = get_param(bh, 'popup_spring_control_A2');
      | 
      | psg_h.Visible  = 'off';
      | 
      | if strcmp(controlParamValue, 'Hydropneumatic')
      |     psg_h.Visible  = 'on';
      | else
      |     psg_h.Visible  = 'off';
      | end
      mask TypeOptions popup_gas_spring_A2: Spring Control A2/popup_gas_spring
  Susp : Subsystem  mask(Steer Control, Two Axle){Steer=Control.Default.Steer}
      mask prompts: Steer "Steer (structure)"
      mask help: Steering control for two-axle vehicles.
  CtrlBus : Outport  VectorParamsAs1DForOutWhenUnconnected=off
  wires:
  Ctrl/1(Ctrl) -> Damper Control/2(Ctrl), Spring Control/2(Ctrl)
  DrvBus/1 -> Bus Selector1/1
  Bus Creator2/1 -> CtrlBus/1  "CtrlBus"
  Bus Selector1/3 -> Brake Control/1("rBrakePedal ")  "<rBrakePedal>"
  Bus Selector1/2 -> Power Control/1(rAccelPedal)  "<rAccelPedal>"
  Spring Control/1(Spring) -> Bus Creator1/4
  Power Control/1(Power) -> Bus Creator2/2
  Driveline Control/1(Driveline) -> Bus Creator2/3
  Damper Control/1(Damper) -> Bus Creator1/3
  Bus Creator1/1 -> Bus Creator2/1  "Chassis"
  Brake Control/1(" Brakes") -> Bus Creator2/4
  Susp/1(SuspA1) -> Bus Creator1/1
  VehBus/1 -> Brake Control/2("VehBus "), Power Control/2(VehBus), Damper Control/1(VehBus), Spring Control/1(VehBus), Bus Selector/1
  Susp/2(SuspA2) -> Bus Creator1/2
  Bus Selector1/1 -> Susp/1(aSteerWheel)  "<aSteerWheel>"
  Bus Selector/1 -> Susp/2(vx)  "<vx>"
  Bus Selector1/4 -> Power Control/3(vTgt)  "<vTarget>"

== system sm_car/Controller/TrqVec 4Motor ==
  DrvBus : Inport
  VehBus : Inport  Port=2
  Brake Control : Subsystem  Variant=on  VariantControlMode=label  VariantControl=Variant1  LabelModeActiveChoice=Pedal  mask{popup_brake_control=Pedal, abs_tire_radiusF=Vehicle.Chassis.TireA1.tire_radius.Value, abs_tire_radiusR=Vehicle.Chassis.TireA2.tire_radius.Value}
      mask prompts: popup_brake_control "Control Type"; abs_tire_radiusF "Tire Radius Front (m)"; abs_tire_radiusR "Tire Radius Rear (m)"
      mask init:
      | set_param(gcb,'LabelModeActiveChoice',get_param(gcb,'popup_brake_control'));
      settings: AttributesFormatString=%<ActiveVariant>
      mask TypeOptions popup_brake_control: Pedal | Pressure | ABS
      mask Display: disp(' ');
  Bus Creator1 : BusCreator  Inputs=4
  Bus Creator2 : BusCreator  Inputs=4
  Bus Selector : BusSelector  OutputSignals=aSteerWheel
  Bus Selector1 : BusSelector  OutputSignals=rBrakePedal
  Bus Selector2 : BusSelector  OutputSignals=Chassis.Body.CG.vx
  Ctrl : Subsystem
  Damper Control : Subsystem  VariantControl=Choice  mask(Damper Control, Two Axle){popup_damper_control_A1=None, popup_damper_control_A2=None}
      mask prompts: popup_damper_control_A1 "Damper Control Axle 1"; popup_damper_control_A2 "Damper Control Axle 2"
      mask help: Configurable damper control for two axles, left and right sides.
      mask TypeOptions popup_damper_control_A1: Damper Control A1/popup_damper_control
      mask TypeOptions popup_damper_control_A2: Damper Control A2/popup_damper_control
  Driveline Control : Subsystem
  Power_TqVec : Subsystem  mask{Control=Control.TrqVec}
      mask prompts: Control "Control Parameters"
  Spring Control : Subsystem  VariantControl=Choice  mask(Spring Control, Two Axles){popup_spring_control_A1=None, popup_gas_spring_A1=Stiff, popup_spring_control_A2=None, popup_gas_spring_A2=Stiff}
      mask prompts: popup_spring_control_A1 "Spring Control Axle 1"; popup_gas_spring_A1 "Gas Spring (Axle 1)"; popup_spring_control_A2 "Spring Control Axle 2"; popup_gas_spring_A2 "Gas Spring (Axle 2)"
      mask help: Configurable spring control for two axles, left and right sides.
      mask TypeOptions popup_spring_control_A1: Spring Control A1/popup_spring_control
      mask Callback popup_spring_control_A1:
      | bh = gcb;
      | maskObj = Simulink.Mask.get(bh); % Get the mask object of the current block
      | psg_h   = maskObj.getParameter('popup_gas_spring_A1'); % Get the parameter to hide
      | 
      | % Check the value of ControlParam
      | controlParamValue = get_param(bh, 'popup_spring_control_A1');
      | 
      | psg_h.Visible  = 'off';
      | 
      | if strcmp(controlParamValue, 'Hydropneumatic')
      |     psg_h.Visible  = 'on';
      | else
      |     psg_h.Visible  = 'off';
      | end
      mask TypeOptions popup_gas_spring_A1: Spring Control A1/popup_gas_spring
      mask TypeOptions popup_spring_control_A2: Spring Control A2/popup_spring_control
      mask Callback popup_spring_control_A2:
      | bh = gcb;
      | maskObj = Simulink.Mask.get(bh); % Get the mask object of the current block
      | psg_h   = maskObj.getParameter('popup_gas_spring_A2'); % Get the parameter to hide
      | 
      | % Check the value of ControlParam
      | controlParamValue = get_param(bh, 'popup_spring_control_A2');
      | 
      | psg_h.Visible  = 'off';
      | 
      | if strcmp(controlParamValue, 'Hydropneumatic')
      |     psg_h.Visible  = 'on';
      | else
      |     psg_h.Visible  = 'off';
      | end
      mask TypeOptions popup_gas_spring_A2: Spring Control A2/popup_gas_spring
  Susp : Subsystem  mask(Steer Control, Two Axle){Steer=Control.Default.Steer}
      mask prompts: Steer "Steer (structure)"
      mask help: Steering control for two-axle vehicles.
  CtrlBus : Outport  VectorParamsAs1DForOutWhenUnconnected=off
  wires:
  Ctrl/1(Ctrl) -> Damper Control/2(Ctrl), Spring Control/2(Ctrl)
  VehBus/1 -> Brake Control/2("VehBus "), Power_TqVec/2(VehBus), Spring Control/1(VehBus), Bus Selector2/1, Damper Control/1(VehBus)
  Bus Selector2/1 -> Susp/2(vx)  "<vx>"
  Bus Selector/1 -> Susp/1(aSteerWheel)  "<aSteerWheel>"
  DrvBus/1 -> Bus Selector/1, Power_TqVec/1(DrvBus), Bus Selector1/1
  Bus Creator2/1 -> CtrlBus/1  "CtrlBus"
  Bus Selector1/1 -> Brake Control/1("rBrakePedal ")  "<rBrakePedal>"
  Spring Control/1(Spring) -> Bus Creator1/4
  Power_TqVec/1(Power) -> Bus Creator2/2
  Driveline Control/1(Driveline) -> Bus Creator2/3
  Damper Control/1(Damper) -> Bus Creator1/3
  Bus Creator1/1 -> Bus Creator2/1  "Chassis"
  Brake Control/1(" Brakes") -> Bus Creator2/4
  Susp/1(SuspA1) -> Bus Creator1/1
  Susp/2(SuspA2) -> Bus Creator1/2

== system sm_car/Driver/Closed Loop ==
  VehBus : Inport
  Obs : Inport  Port=2
  Bus Selector2 : BusSelector  OutputSignals=dist
  Driver : Subsystem  mask(Driver Behavior){Driver=Driver}
      mask help: Models driver behavior to follow prescribed vehicle trajectory, including path and speed.
  Driver Override : Subsystem  Variant=on  VariantControlMode=label  VariantControl=Choice  LabelModeActiveChoice=None  mask(Override Driver Commands){popup_driver_override=None}
      mask prompts: popup_driver_override "Driver Override"
      mask help: Override closed-loop driver commands with open-loop inputs. Can be applied to steering wheel, accelerator pedal. or brake pedal.
      mask init:
      | curblk = gcb;
      | 
      | set_param(curblk,'LabelModeActiveChoice',get_param(curblk,'popup_driver_override'));
      mask TypeOptions popup_driver_override: None | Override
  Maneuver : Subsystem  mask(Maneuver Follow Trajectory){Maneuver=Maneuver, popup_window=No}
      mask prompts: popup_window "Check only window of trajectory"
      mask help: Determines target pose to follow prescribed trajectory. Prescribed trajectory is vehicle pose (x, y, theta) and speed along the path to be followed. Optional visual of target pose is also provided.
      mask init:
      | if(strcmpi(get_param(gcb,'popup_window'),'yes'))
      |     set_param([gcb '/window only'],'Value','1');
      | else
      |     set_param([gcb '/window only'],'Value','0');
      | end
      mask TypeOptions popup_window: No | Yes
  Override : Subsystem  Variant=on  VariantControlMode=label  VariantControl=Variant1  LabelModeActiveChoice=None  mask(Driver Override){popup_override_type=None}
      mask prompts: popup_override_type "Override Type"
      mask help: Optionally override driver commands based on objects in scene. For example, the state of a traffic light can override driver commands to follow a prescribed speed trajectory.
      mask init:
      | set_param(gcb,'LabelModeActiveChoice',strrep(get_param(gcb,'popup_override_type'),' ','_'));
      settings: AttributesFormatString=%<LabelModeActiveChoice>
      mask TypeOptions popup_override_type: None | Track Mallory Park Obstacle
      mask Display: disp(' ');
  Scopes : Subsystem
  Terminator : Terminator
  Transfer Fcn : TransferFcn  Denominator=[0.1 1]
  DrvBus : Outport  VectorParamsAs1DForOutWhenUnconnected=off
  wires:
  Driver Override/1(DrvBus) -> DrvBus/1
  Maneuver/3(CurPose) -> Driver/3(CurPose), Scopes/3(CurPose)
  VehBus/1 -> Maneuver/1(VehBus)
  Maneuver/4(Preview) -> Driver/4(Preview)
  Driver/1(DrvBus) -> Driver Override/1(In), Scopes/4(DrvBus)
  Obs/1 -> Override/2("Obs ")
  Bus Selector2/1 -> Transfer Fcn/1  "<dist>"
  Override/1(" Ovr") -> Maneuver/2(Override)
  Transfer Fcn/1 -> Override/1("dist ")
  Maneuver/5(simres) -> Terminator/1
  Maneuver/1(vx) -> Driver/1(vx), Scopes/1(<vx>)
  Maneuver/2(Ref) -> Driver/2(Ref), Scopes/2(Ref), Bus Selector2/1

== system sm_car/Driver/Open Loop ==
  VehBus : Inport
  Obs : Inport  Port=2
  Open Loop : Subsystem  mask{Maneuver=Maneuver}
      mask init:
      | X = [0 0];
      | Y = [0 0];
  Terminator : Terminator
  Terminator1 : Terminator
  DrvBus : Outport  VectorParamsAs1DForOutWhenUnconnected=off
  wires:
  Obs/1 -> Terminator1/1
  VehBus/1 -> Terminator/1
  Open Loop/1(DrvBus) -> DrvBus/1

== system sm_car/Road/Ground ==
  gz : Inport
  uvec : Inport  Port=2
  fcp : Inport  Port=3
  fco : Inport  Port=4
  fwc : Inport  Port=5
  TyreScaling FL : Inport  Port=6
  TyreScaling FR : Inport  Port=7
  TyreScaling RL : Inport  Port=8
  TyreScaling RR : Inport  Port=9
  Bus Creator{,1..3} (4 alike) : BusCreator  Inputs=6
  Bus Selector : BusSelector  OutputSignals=L1,R1,L2,R2
  Bus Selector1 : BusSelector  OutputSignals=L1,R1,L2,R2
  Bus Selector2 : BusSelector  OutputSignals=L1.fx,L1.fy,L1.tz  OutputAsBus=on
  Bus Selector3 : BusSelector  OutputSignals=R1.fx,R1.fy,R1.tz  OutputAsBus=on
  Bus Selector4 : BusSelector  OutputSignals=L2.fx,L2.fy,L2.tz  OutputAsBus=on
  Bus Selector5 : BusSelector  OutputSignals=R2.fx,R2.fy,R2.tz  OutputAsBus=on
  Bus Selector6 : BusSelector  OutputSignals=L1.fcoy,R1.fcoy,L2.fcoy,R2.fcoy
  Bus Selector7 : BusSelector  OutputSignals=L1.fwcx,R1.fwcx,L2.fwcx,R2.fwcx
  Gain{,1..7} (8 alike) : Gain
  Signal Specification1 : SignalSpecification  Unit=m
  L1 : Outport  VectorParamsAs1DForOutWhenUnconnected=off
  R1 : Outport  Port=2  VectorParamsAs1DForOutWhenUnconnected=off
  L2 : Outport  Port=3  VectorParamsAs1DForOutWhenUnconnected=off
  R2 : Outport  Port=4  VectorParamsAs1DForOutWhenUnconnected=off
  wires:
  Bus Creator/1 -> L1/1  "L1"
  Bus Creator1/1 -> R1/1  "R1"
  Gain1/1 -> Bus Creator1/1  "gz"
  TyreScaling FL/1 -> Bus Creator/3  "TyreScaling"
  Bus Creator3/1 -> R2/1  "R2"
  gz/1 -> Signal Specification1/1
  Gain3/1 -> Bus Creator3/1  "gz"
  Bus Creator2/1 -> L2/1  "L2"
  Signal Specification1/1 -> Bus Selector/1
  Gain2/1 -> Bus Creator2/1  "gz"
  TyreScaling FR/1 -> Bus Creator1/3  "TyreScaling"
  TyreScaling RL/1 -> Bus Creator2/3  "TyreScaling"
  TyreScaling RR/1 -> Bus Creator3/3  "TyreScaling"
  Bus Selector/1 -> Gain/1  "<L1>"
  Gain/1 -> Bus Creator/1  "gz"
  Bus Selector/2 -> Gain1/1  "<R1>"
  Bus Selector/3 -> Gain2/1  "<L2>"
  Bus Selector/4 -> Gain3/1  "<R2>"
  uvec/1 -> Bus Selector1/1
  Bus Selector1/1 -> Gain4/1  "<L1>"
  Bus Selector1/2 -> Gain5/1  "<R1>"
  Bus Selector1/3 -> Gain6/1  "<L2>"
  Bus Selector1/4 -> Gain7/1  "<R2>"
  Gain4/1 -> Bus Creator/2  "uvec"
  Gain5/1 -> Bus Creator1/2  "uvec"
  Gain6/1 -> Bus Creator2/2  "uvec"
  Gain7/1 -> Bus Creator3/2  "uvec"
  fcp/1 -> Bus Selector5/1, Bus Selector4/1, Bus Selector3/1, Bus Selector2/1
  Bus Selector2/1 -> Bus Creator/4  "fcp"
  Bus Selector3/1 -> Bus Creator1/4  "fcp"
  Bus Selector4/1 -> Bus Creator2/4  "fcp"
  Bus Selector5/1 -> Bus Creator3/4  "fcp"
  fco/1 -> Bus Selector6/1
  Bus Selector6/1 -> Bus Creator/5  "<fcoy>"
  Bus Selector6/2 -> Bus Creator1/5  "<fcoy>"
  Bus Selector6/3 -> Bus Creator2/5  "<fcoy>"
  Bus Selector6/4 -> Bus Creator3/5  "<fcoy>"
  fwc/1 -> Bus Selector7/1
  Bus Selector7/1 -> Bus Creator/6  "<fwcx>"
  Bus Selector7/2 -> Bus Creator1/6  "<fwcx>"
  Bus Selector7/3 -> Bus Creator2/6  "<fwcx>"
  Bus Selector7/4 -> Bus Creator3/6  "<fwcx>"

== system sm_car/Road/Input fWindCar ==
  Bus Creator1 : BusCreator  Inputs=3
  Demux : Demux  Outputs=3
  Step : Step  Time=dWind  After=fWind  SampleTime=0
  Step1 : Step  Time=dWind+tWind  After=fWind  SampleTime=0
  Sum : Sum  Inputs=|+-
  fWind : Outport  VectorParamsAs1DForOutWhenUnconnected=off
  wires:
  Demux/2 -> Bus Creator1/2  "fy"
  Demux/1 -> Bus Creator1/1  "fx"
  Demux/3 -> Bus Creator1/3  "fz"
  Bus Creator1/1 -> fWind/1
  Step/1 -> Sum/1
  Step1/1 -> Sum/2
  Sum/1 -> Demux/1

== system sm_car/Road/Input fWindTrailer ==
  Bus Creator1 : BusCreator  Inputs=3
  Demux : Demux  Outputs=3
  Scope : Scope
      settings: ActiveDisplayYMinimum=-1  ActiveDisplayYMaximum=1
  Step : Step  Time=dWind  After=fWind  SampleTime=0
  Step1 : Step  Time=dWind+tWind  After=fWind  SampleTime=0
  Sum : Sum  Inputs=|+-
  fWind : Outport  VectorParamsAs1DForOutWhenUnconnected=off
  wires:
  Bus Creator1/1 -> fWind/1
  Demux/3 -> Bus Creator1/3  "fz"
  Demux/1 -> Bus Creator1/1  "fx"
  Demux/2 -> Bus Creator1/2  "fy"
  Sum/1 -> Scope/1, Demux/1  "fxyz"
  Step1/1 -> Sum/2
  Step/1 -> Sum/1
